simulink model "Seven_Level_inverter_Asymmetrical"  (R2025a)
settings: Solver=VariableStepAuto  StartTime=0.0  StopTime=10  RelTol=1e-3
undefined symbols (not defined in the file): fc, Ts
libraries: spsIGBTDiodeLib x8, simulink x6, spsDCVoltageSourceLib x2, spsSeriesRLCBranchLib x1, spsVoltageMeasurementLib x1, sps_lib x1
settings Model: Creator=HP  LastModifiedBy=HP

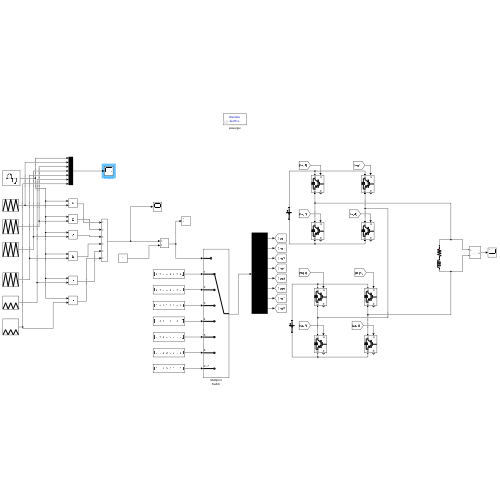
[thumbnail: Simulink's stored preview of the top-level diagram]
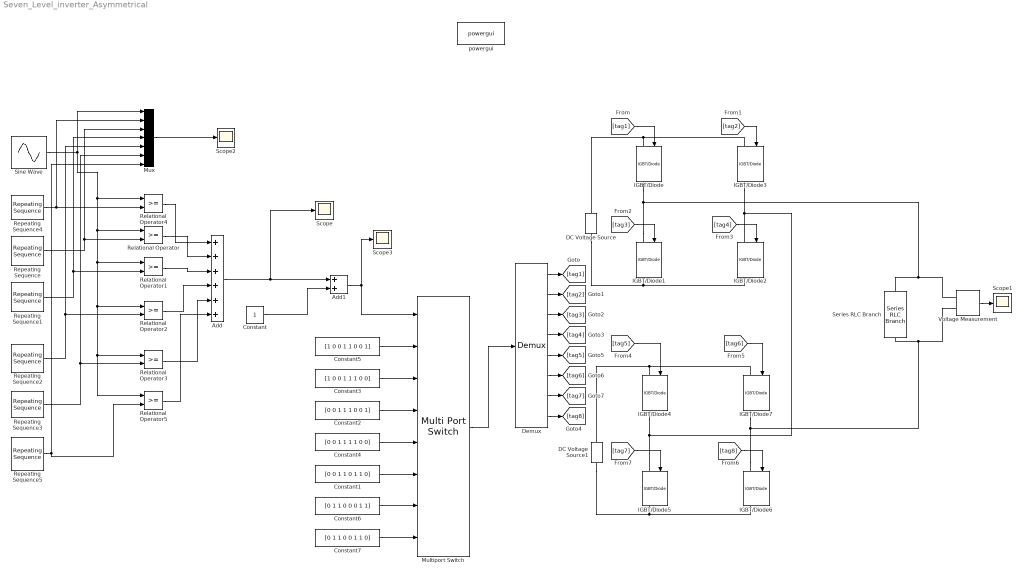
== system Seven_Level_inverter_Asymmetrical ==
  Add : Sum  Inputs=++++++
  Add1 : Sum
  Constant : Constant
  Constant1 : Constant  Value=[0 0 1 1 0 1 1 0]
  Constant2 : Constant  Value=[0 0 1 1 1 0 0 1]
  Constant3 : Constant  Value=[1 0 0 1 1 1 0 0]
  Constant4 : Constant  Value=[0 0 1 1 1 1 0 0]
  Constant5 : Constant  Value=[1 0 0 1 1 0 0 1]
  Constant6 : Constant  Value=[0 1 1 0 0 0 1 1]
  Constant7 : Constant  Value=[0 1 1 0 0 1 1 0]
  DC Voltage Source : spsDCVoltageSourceLib/DC Voltage Source  Amplitude=200  Measurements=None
  DC Voltage Source1 : spsDCVoltageSourceLib/DC Voltage Source  Amplitude=100  Measurements=None
  Demux : Demux  Outputs=8
  IGBT/Diode{,1..7} (8 alike) : spsIGBTDiodeLib/IGBT//Diode  Ron=1e-3  Rs=1e5  Cs=inf  Measurements=on
  Multiport Switch : MultiPortSwitch  Inputs=7  SaturateOnIntegerOverflow=off  InputSameDT=off
  Mux : Mux  Inputs=7
  Relational Operator{,1..5} (6 alike) : RelationalOperator  OutDataTypeStr=boolean  RndMeth=Simplest  InputSameDT=off
  Repeating Sequence : simulink/Sources/Repeating Sequence  rep_seq_t=[0 0.5/fc 1/fc]  rep_seq_y=[1 2 1]
  Repeating Sequence1 : simulink/Sources/Repeating Sequence  rep_seq_t=[0 0.5/fc 1/fc]  rep_seq_y=[0 1 0]
  Repeating Sequence2 : simulink/Sources/Repeating Sequence  rep_seq_t=[0 0.5/fc 1/fc]  rep_seq_y=[-1 0 -1]
  Repeating Sequence3 : simulink/Sources/Repeating Sequence  rep_seq_t=[0 0.5/fc 1/fc]  rep_seq_y=[-2 -1 -2]
  Repeating Sequence4 : simulink/Sources/Repeating Sequence  rep_seq_t=[0 0.5/fc 1/fc]  rep_seq_y=[2 3 2]
  Repeating Sequence5 : simulink/Sources/Repeating Sequence  rep_seq_t=[0 0.5/fc 1/fc]  rep_seq_y=[-3 -2 -3]
  Scope{,1..3} (4 alike) : Scope
      Scope settings: ActiveDisplayYMinimum=-0.74999999999999978  ActiveDisplayYMaximum=6.75
      Scope1 settings: ActiveDisplayYMinimum=-375.06272847741695  ActiveDisplayYMaximum=375.06163974721665
      Scope2 settings: ActiveDisplayYMinimum=-3.7374999999999985  ActiveDisplayYMaximum=3.6374999999999873  DataLoggingVariableName=ScopeData2
      Scope3 settings: ActiveDisplayYMinimum=0.25000000000000022  ActiveDisplayYMaximum=7.75  DataLoggingVariableName=ScopeData3
  Series RLC Branch : spsSeriesRLCBranchLib/Series RLC Branch  LConnTagsString=__new0  RConnTagsString=__new0  BranchType=RL  Resistance=1  Inductance=0.1  SetiL0=off  InitialCurrent=0  Capacitance=1e-6  Setx0=off  InitialVoltage=0  Measurements=None
  Sine Wave : Sin  Amplitude=2.9  Frequency=2*pi*50  SampleTime=Ts
  Voltage Measurement : spsVoltageMeasurementLib/Voltage Measurement  PhasorSimulation=off  OutputType=Complex  PSBequivalent=0
  powergui : sps_lib/powergui  Priority=1  SimulationMode=Discrete  SampleTime=20e-6  frequency=60  Iterations=50  frequencyindice=0  Pbase=100e6  ErrMax=1e-4  UnitsV=kV  UnitsW=MW  buscounter=0  FunctionMessages=off  echomessages=off  EnableUseOfTLC=off  CurrentSourceSwitches=off  DisableSnubberDevices=off  DisableRonSwitches=off  DisableVfSwitches=off  DisplayEquations=off  AutomaticDiscreteSolvers=off  SolverType=Tustin/Backward Euler (TBE)  Interpol=off  ExternalGateDelay=off  methode=off  Ts=100  x0status=blocks  SPID=on  SwTol=0  HookPort=off  NonlinearTolerance=1e-4  nMaxIteration=100  ContinueOnMaxIteration=off  RestoreLinks=warning  ResistiveCurrentMeasurement=off  Frange=[0:2:500]  Ylog=off  Xlog=on  ShowGrid=off  save=off  variable=ZData  structure=0  ZoomFFT=off  StartTime=0.0  cycles=1  DisplayStyle=1  fundamental=60  FreqAxis=off  MaxFrequency=1000  frequencyindicesteady=1  RmsSteady=1  display=off
  wires:
  Repeating Sequence2/1 -> Mux/5, Relational Operator2/2
  Constant6/1 -> Multiport Switch/7
  [tag3] -> IGBT/Diode1/1
  [tag6] -> IGBT/Diode7/1
  Constant/1 -> Add1/2
  Relational Operator2/1 -> Add/4
  Repeating Sequence5/1 -> Relational Operator5/2, Mux/7
  Demux/3 -> [tag3]
  Relational Operator3/1 -> Add/5
  Relational Operator4/1 -> Add/1
  [tag2] -> IGBT/Diode3/1
  Repeating Sequence3/1 -> Mux/6, Relational Operator3/2
  Repeating Sequence1/1 -> Mux/4, Relational Operator1/2
  Demux/4 -> [tag4]
  Sine Wave/1 -> Relational Operator4/1, Relational Operator5/1, Relational Operator3/1, Relational Operator2/1, Relational Operator1/1, Relational Operator/1, Mux/1
  Demux/6 -> [tag6]
  [tag1] -> IGBT/Diode/1
  Mux/1 -> Scope2/1
  Constant5/1 -> Multiport Switch/2
  [tag4] -> IGBT/Diode2/1
  Multiport Switch/1 -> Demux/1
  Demux/8 -> [tag8]
  Constant3/1 -> Multiport Switch/3
  Add1/1 -> Scope3/1, Multiport Switch/1
  Repeating Sequence/1 -> Mux/3, Relational Operator/2
  Constant7/1 -> Multiport Switch/8
  Constant2/1 -> Multiport Switch/4
  Demux/7 -> [tag7]
  Constant1/1 -> Multiport Switch/6
  Constant4/1 -> Multiport Switch/5
  Add/1 -> Scope/1, Add1/1
  Demux/2 -> [tag2]
  [tag7] -> IGBT/Diode5/1
  Relational Operator/1 -> Add/2
  Repeating Sequence4/1 -> Mux/2, Relational Operator4/2
  [tag5] -> IGBT/Diode4/1
  Relational Operator5/1 -> Add/6
  [tag8] -> IGBT/Diode6/1
  Demux/5 -> [tag5]
  Relational Operator1/1 -> Add/3
  Demux/1 -> [tag1]
  Voltage Measurement/1 -> Scope1/1
  connections:
  IGBT/Diode2/RConn1 -- IGBT/Diode1/RConn1 -- DC Voltage Source/LConn1
  IGBT/Diode1/LConn1 -- Series RLC Branch/LConn1 -- Voltage Measurement/LConn1 -- IGBT/Diode/RConn1
  IGBT/Diode4/RConn1 -- IGBT/Diode5/LConn1 -- IGBT/Diode2/LConn1 -- IGBT/Diode3/RConn1
  IGBT/Diode7/LConn1 -- IGBT/Diode4/LConn1 -- DC Voltage Source1/RConn1
  IGBT/Diode6/RConn1 -- IGBT/Diode5/RConn1 -- DC Voltage Source1/LConn1
  IGBT/Diode3/LConn1 -- IGBT/Diode/LConn1 -- DC Voltage Source/RConn1
  IGBT/Diode6/LConn1 -- Series RLC Branch/RConn1 -- Voltage Measurement/LConn2 -- IGBT/Diode7/RConn1
